simulink model "myFirstController_sim"  (R2012b)
settings: Solver=ode45  StartTime=0.0  StopTime=15  RelTol=1e-3
undefined symbols (not defined in the file or in its folder): A, B, C_all
settings Model: Creator=Juan  LastModifiedBy=juanj
settings DataIOCC: SignalLoggingSaveFormat=ModelDataLogs
settings OptimizationCC: ExpressionDepthLimit=128
settings DebuggingCC: MultiTaskDSMMsg=warning  MultiTaskCondExecSysMsg=none  StrictBusMsg=None
settings RTWCC: IncludeERTFirstTime=on
settings CodeAppCC: CustomSymbolStrType=$N$R$M_T  InternalIdentifier=Shortened

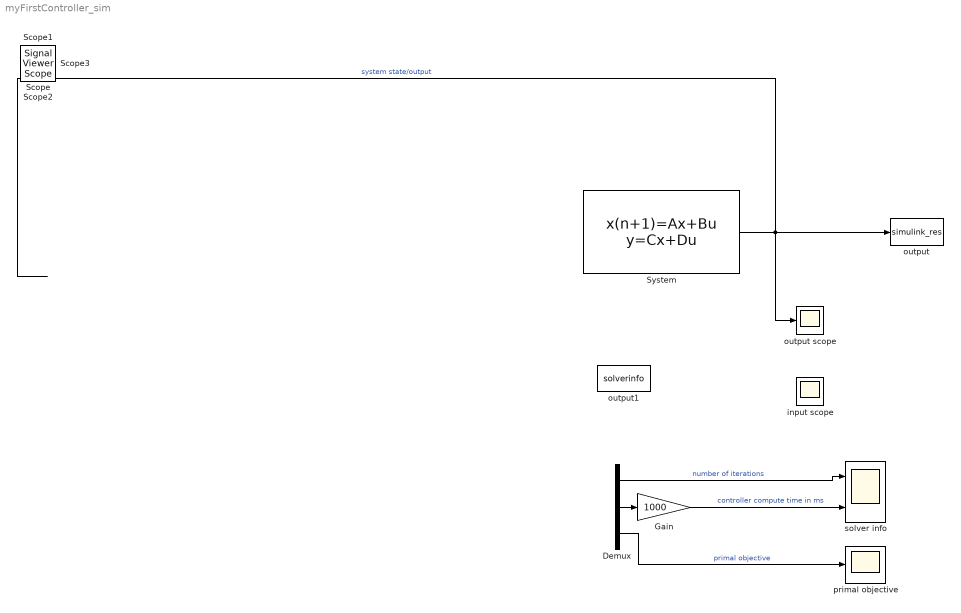
== system myFirstController_sim ==
  Demux : Demux  Outputs=3
  Gain : Gain  Gain=1000
  System : DiscreteStateSpace  A=A  B=B  C=C_all  D=zeros(2,1)  X0=[0; 6]
  input scope : Scope
      settings: TimeRange=140  YMin=-26  YMax=26  SaveName=ScopeData4
  output : ToWorkspace  VariableName=simulink_res  SampleTime=-1  SaveFormat=Timeseries
  output scope : Scope
      settings: TimeRange=140  YMin=-26  YMax=26
  output1 : ToWorkspace  VariableName=solverinfo  SampleTime=-1  SaveFormat=Timeseries
  primal objective : Scope
      settings: TimeRange=140  YMin=-26  YMax=26  SaveName=ScopeData3
  solver info : Scope  NumInputPorts=2
      settings: TimeRange=140  YMin=22~0.9  YMax=26~1.6  SaveName=ScopeData2
  Scope : SignalViewerScope  IOType=viewer  ZoomMode=yonly  RefreshTime=0.035000
      settings: YMin=-25  YMax=25
  Scope1 : SignalViewerScope  IOType=viewer  RefreshTime=0.035000
  Scope2 : SignalViewerScope  IOType=viewer  RefreshTime=0.035000
      settings: SaveName=ScopeData2
  Scope3 : SignalViewerScope  IOType=viewer  RefreshTime=0.035000
      settings: SaveName=ScopeData3
  wires:
  System/1 -> output scope/1, output/1  "system state/output"
  ? -> input scope/1, System/1  "optimal input"
  ? -> Demux/1, output1/1  "solver info"
  Demux/2 -> Gain/1
  Gain/1 -> solver info/2  "controller compute time in ms"
  Demux/1 -> solver info/1  "number of iterations"
  Demux/3 -> primal objective/1  "primal objective"
